simulink model "FMS"  (R2018b)
settings: configuration reference "fms_config" (kept outside this file)
values from neighbouring files (symbols this model uses):
  FMS_EXPORT = Simulink.Parameter(FMS_EXPORT_VALUE)    [fms_model_init.m]
  FMS_PARAM = Simulink.Parameter(FMS_PARAM_VALUE)    [fms_model_init.m]
undefined symbols (not defined in the file or in its folder): actuator_cmd, ay_cmd, cmd_mask, ControlMode, ctrl_mode, DiscIntNeverNeededParam, FMS_Cmd, mode, PilotMode, r_cmd, reset, state, status, theta_cmd, timestamp, u_cmd, VehicleState, VehicleStatus, w_cmd, wp_consume, wp_current
libraries: simulink x27, FMT_Model_Lib x21, hdlsllib x4
(part 1 of 3)
settings Model: Creator=jc  LastModifiedBy=zouji
settings ConfigSetRef: SourceLocation=Base Workspace

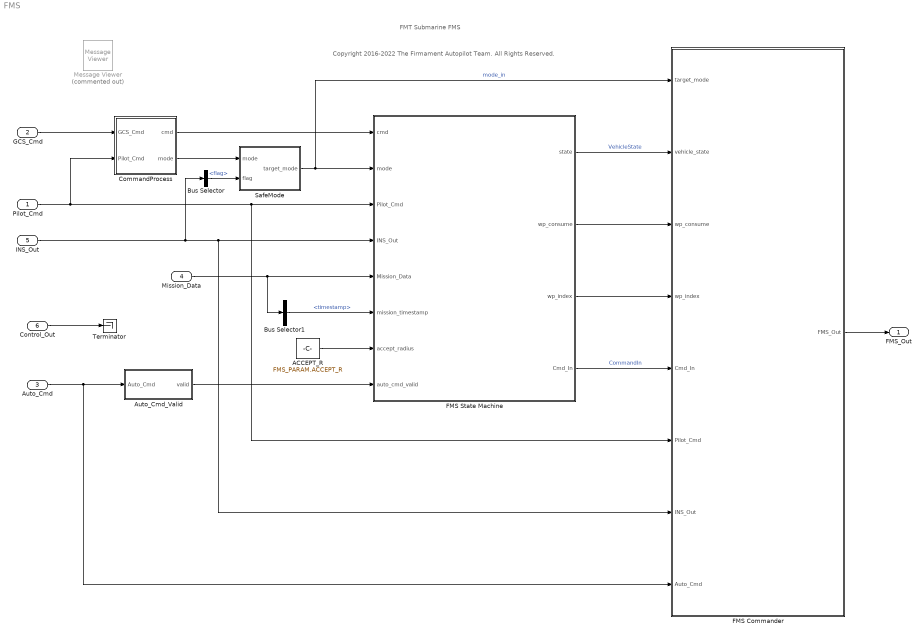
== system FMS ==
  note: Copyright 2016-2022 The Firmament Autopilot Team. All Rights Reserved.
  note: FMT Submarine FMS
  Pilot_Cmd : Inport  OutDataTypeStr=Bus: Pilot_Cmd_Bus
  GCS_Cmd : Inport  Port=2  OutDataTypeStr=Bus: GCS_Cmd_Bus
  Auto_Cmd : Inport  Port=3  OutDataTypeStr=Bus: Auto_Cmd_Bus
  Mission_Data : Inport  Port=4  OutDataTypeStr=Bus: Mission_Data_Bus  BusOutputAsStruct=on
  INS_Out : Inport  Port=5  OutDataTypeStr=Bus: INS_Out_Bus
  Control_Out : Inport  Port=6  OutDataTypeStr=Bus: Control_Out_Bus
  ACCEPT_R : Constant  Value=FMS_PARAM.ACCEPT_R
  Auto_Cmd_Valid : Subsystem
  Bus Selector : BusSelector  OutputSignals=flag
  Bus Selector1 : BusSelector  OutputSignals=timestamp
  CommandProcess : Subsystem  TreatAsAtomicUnit=on
  FMS Commander : Subsystem  TreatAsAtomicUnit=on
  FMS State Machine : Stateflow chart  TreatAsAtomicUnit=on
  Message Viewer : MessageViewer  Commented=on  SavedRootId=#
  SafeMode : Stateflow chart  TreatAsAtomicUnit=on
  Terminator : Terminator
  FMS_Out : Outport  OutDataTypeStr=Bus: FMS_Out_Bus
  wires:
  Control_Out/1 -> Terminator/1
  CommandProcess/1(cmd) -> FMS State Machine/1(cmd)
  FMS State Machine/4(Cmd_In) -> FMS Commander/5(Cmd_In)  "CommandIn"
  Auto_Cmd/1 -> Auto_Cmd_Valid/1(Auto_Cmd), FMS Commander/8(Auto_Cmd)
  Pilot_Cmd/1 -> FMS Commander/6(Pilot_Cmd), FMS State Machine/3(Pilot_Cmd), CommandProcess/2(Pilot_Cmd)
  INS_Out/1 -> Bus Selector/1, FMS Commander/7(INS_Out), FMS State Machine/4(INS_Out)
  CommandProcess/2(mode) -> SafeMode/1(mode)
  FMS Commander/1(FMS_Out) -> FMS_Out/1
  Bus Selector/1 -> SafeMode/2(flag)  "<flag>"
  GCS_Cmd/1 -> CommandProcess/1(GCS_Cmd)
  SafeMode/1(target_mode) -> FMS Commander/1(target_mode), FMS State Machine/2(mode)  "mode_in"
  FMS State Machine/1(state) -> FMS Commander/2(vehicle_state)  "VehicleState"
  Mission_Data/1 -> Bus Selector1/1, FMS State Machine/5(Mission_Data)
  FMS State Machine/2(wp_consume) -> FMS Commander/3(wp_consume)
  Bus Selector1/1 -> FMS State Machine/6(mission_timestamp)  "<timestamp>"
  FMS State Machine/3(wp_index) -> FMS Commander/4(wp_index)
  ACCEPT_R/1 -> FMS State Machine/7(accept_radius)
  Auto_Cmd_Valid/1(valid) -> FMS State Machine/8(auto_cmd_valid)

== system FMS/Auto_Cmd_Valid ==
  Auto_Cmd : Inport
  Bus Selector1 : BusSelector  OutputSignals=frame
  Bus Selector2 : BusSelector  OutputSignals=timestamp
  Compare To Constant4 : simulink/Logic and Bit Operations/Compare To Constant  relop=<  const=1000  OutDataTypeStr=boolean
  Constant : Constant  Value=FMS_EXPORT.period  OutDataTypeStr=single
  Detect Change : simulink/Logic and Bit Operations/Detect Change  vinit=0  OutDataTypeStr=boolean
  Discrete-Time Integrator : DiscreteIntegrator  IntegratorMethod=Accumulation: Forward Euler  ExternalReset=sampled level  SampleTime=-1  OutDataTypeStr=uint32  SaturateOnIntegerOverflow=on  ICPrevOutput=DiscIntNeverNeededParam  ICPrevScaledInput=DiscIntNeverNeededParam
  Ever_Valid : Subsystem
  Interval Test : simulink/Logic and Bit Operations/Interval Test  IntervalClosedRight=on  uplimit=2  IntervalClosedLeft=on  lowlimit=0  OutDataTypeStr=boolean
  Logical Operator : Logic  Inputs=3  AllPortsSameDT=off  OutDataTypeStr=boolean
  valid : Outport
  wires:
  Constant/1 -> Discrete-Time Integrator/1
  Detect Change/1 -> Ever_Valid/1(in), Discrete-Time Integrator/2
  Discrete-Time Integrator/1 -> Compare To Constant4/1
  Auto_Cmd/1 -> Bus Selector1/1, Bus Selector2/1
  Compare To Constant4/1 -> Logical Operator/1
  Ever_Valid/1(out) -> Logical Operator/2
  Logical Operator/1 -> valid/1
  Bus Selector2/1 -> Detect Change/1  "<timestamp>"
  Bus Selector1/1 -> Interval Test/1  "<frame>"
  Interval Test/1 -> Logical Operator/3

== system FMS/CommandProcess ==
  GCS_Cmd : Inport
  Pilot_Cmd : Inport  Port=2
  Check Valid : Subsystem
  Command Routing : Subsystem
  Mode Routing : Subsystem
  cmd : Outport
  mode : Outport  Port=2
  wires:
  GCS_Cmd/1 -> Mode Routing/2(GCS_Cmd), Command Routing/1(gcs_cmd)
  Pilot_Cmd/1 -> Command Routing/2(pilot_cmd), Check Valid/1(Pilot_Cmd), Mode Routing/3(Pilot_Cmd)
  Command Routing/1(cmd) -> cmd/1
  Check Valid/1(pilot_cmd_valid) -> Mode Routing/1(pilot_cmd_valid)
  Mode Routing/1(mode) -> mode/1  "fms_mode"

== system FMS/FMS Commander ==
  target_mode : Inport
  vehicle_state : Inport  Port=2
  wp_consume : Inport  Port=3
  wp_index : Inport  Port=4
  Cmd_In : Inport  Port=5
  Pilot_Cmd : Inport  Port=6
  INS_Out : Inport  Port=7
  Auto_Cmd : Inport  Port=8
  Commander : Subsystem
  FMS_Input : Subsystem  TreatAsAtomicUnit=on
  FMS_Out : Outport
  wires:
  target_mode/1 -> Commander/1(target_mode)
  FMS_Input/1(FMS_In) -> Commander/2(FMS_In)  "FMS_In"
  Commander/1(FMS_Out) -> FMS_Out/1
  vehicle_state/1 -> FMS_Input/1(state)
  wp_consume/1 -> FMS_Input/2(wp_consume)
  wp_index/1 -> FMS_Input/3(wp_index)
  Cmd_In/1 -> FMS_Input/4(Cmd_In)
  Pilot_Cmd/1 -> FMS_Input/5(Pilot_Cmd)
  INS_Out/1 -> FMS_Input/6(INS_Out)
  Auto_Cmd/1 -> FMS_Input/7(Auto_Cmd)

== system FMS/FMS State Machine/Vehicle.Arm.Auto.Mission.LLA2FLAT ==
  lla : Inport  OutDataTypeStr=double  PortDimensions=[1 3]
  llo : Inport  Port=2  OutDataTypeStr=double  Unit=deg  PortDimensions=[1 2]
  href : Inport  Port=3  OutDataTypeStr=double  Unit=m  PortDimensions=1
  psio : Inport  Port=4  OutDataTypeStr=double  Unit=deg  PortDimensions=1
  f : TriggerPort  TriggerType=function-call  VariantControl=(inherit)
      settings: CopyFcn=Stateflow.SLINSF.SimulinkMan.removeBlockPreDeleteFcn  PreDeleteFcn=Stateflow.SLINSF.SimulinkMan.unsafePredeleteFcn
  Data Type Conversion : DataTypeConversion  OutDataTypeStr=single
  LLA2FLAT : FMT_Model_Lib/Transformation/LLA2FLAT
      settings: SourceProductName=FMT Toolbox
  Signal Conversion : SignalConversion  OverrideOpt=off
  pos : Outport
  wires:
  LLA2FLAT/1 -> Signal Conversion/1
  lla/1 -> LLA2FLAT/1
  llo/1 -> LLA2FLAT/2
  href/1 -> LLA2FLAT/3
  psio/1 -> LLA2FLAT/4
  Signal Conversion/1 -> Data Type Conversion/1
  Data Type Conversion/1 -> pos/1

== system FMS/FMS State Machine/Vehicle.StickMoved ==
  stick_val : Inport  OutDataTypeStr=double  PortDimensions=4
  pilot_cmd : Inport  Port=2  OutDataTypeStr=Bus: Pilot_Cmd_Bus  PortDimensions=1
  f : TriggerPort  TriggerType=function-call  VariantControl=(inherit)
      settings: CopyFcn=Stateflow.SLINSF.SimulinkMan.removeBlockPreDeleteFcn  PreDeleteFcn=Stateflow.SLINSF.SimulinkMan.unsafePredeleteFcn
  Abs : Abs
  Bus Selector : BusSelector  OutputSignals=stick_yaw,stick_throttle,stick_roll,stick_pitch
  Compare To Constant : simulink/Logic and Bit Operations/Compare To Constant  relop=>=  const=0.1  OutDataTypeStr=boolean
  Max : MinMax  Function=max
  Mux : Mux
  Sum : Sum  Inputs=|+-
  moved : Outport
  wires:
  pilot_cmd/1 -> Bus Selector/1
  Bus Selector/1 -> Mux/1  "<stick_yaw>"
  Bus Selector/2 -> Mux/2  "<stick_throttle>"
  Bus Selector/3 -> Mux/3  "<stick_roll>"
  Bus Selector/4 -> Mux/4  "<stick_pitch>"
  stick_val/1 -> Sum/1
  Mux/1 -> Sum/2
  Sum/1 -> Abs/1
  Abs/1 -> Max/1
  Max/1 -> Compare To Constant/1
  Compare To Constant/1 -> moved/1

== system FMS/Auto_Cmd_Valid/Ever_Valid ==
  in : Inport
  Constant1 : Constant  OutDataTypeStr=uint8
  Delay : Delay  DelayLength=1
  Switch : Switch  Criteria=u2 > Threshold
  out : Outport
  wires:
  Constant1/1 -> Switch/1
  Delay/1 -> Switch/3
  in/1 -> Switch/2
  Switch/1 -> out/1, Delay/1

== system FMS/CommandProcess/Check Valid ==
  Pilot_Cmd : Inport
  Bus Selector1 : BusSelector  OutputSignals=timestamp
  Compare To Constant1 : simulink/Logic and Bit Operations/Compare To Constant  relop=<  const=500  OutDataTypeStr=boolean
  Constant1 : Constant  Value=FMS_EXPORT.period  OutDataTypeStr=single
  Detect Change1 : simulink/Logic and Bit Operations/Detect Change  vinit=0  OutDataTypeStr=boolean
  Discrete-Time Integrator1 : DiscreteIntegrator  IntegratorMethod=Accumulation: Forward Euler  ExternalReset=sampled level  SampleTime=-1  OutDataTypeStr=uint32  SaturateOnIntegerOverflow=on  ICPrevOutput=DiscIntNeverNeededParam  ICPrevScaledInput=DiscIntNeverNeededParam
  pilot_cmd_valid : Outport
  wires:
  Pilot_Cmd/1 -> Bus Selector1/1
  Compare To Constant1/1 -> pilot_cmd_valid/1
  Bus Selector1/1 -> Detect Change1/1  "<timestamp>"
  Constant1/1 -> Discrete-Time Integrator1/1
  Detect Change1/1 -> Discrete-Time Integrator1/2
  Discrete-Time Integrator1/1 -> Compare To Constant1/1

== system FMS/CommandProcess/Command Routing ==
  gcs_cmd : Inport
  pilot_cmd : Inport  Port=2
  Bus Selector : BusSelector  OutputSignals=cmd_1
  Bus Selector1 : BusSelector  OutputSignals=cmd_1
  Constant1 : Constant  Value=FMS_Cmd.None
  Data Type Conversion1 : DataTypeConversion  OutDataTypeStr=Enum: FMS_Cmd
  Data Type Conversion2 : DataTypeConversion  OutDataTypeStr=Enum: FMS_Cmd
  Detect Change3 : simulink/Logic and Bit Operations/Detect Change  vinit=0  OutDataTypeStr=boolean
  Detect Change4 : simulink/Logic and Bit Operations/Detect Change  vinit=0  OutDataTypeStr=boolean
  Switch1 : Switch  Criteria=u2 > Threshold
  Switch2 : Switch  Criteria=u2 > Threshold
  cmd : Outport
  wires:
  Bus Selector/1 -> Data Type Conversion1/1, Detect Change4/1  "<cmd_1>"
  pilot_cmd/1 -> Bus Selector1/1
  Switch1/1 -> cmd/1
  gcs_cmd/1 -> Bus Selector/1
  Bus Selector1/1 -> Data Type Conversion2/1, Detect Change3/1  "<cmd_1>"
  Detect Change3/1 -> Switch1/2
  Switch2/1 -> Switch1/3
  Detect Change4/1 -> Switch2/2
  Data Type Conversion2/1 -> Switch1/1
  Data Type Conversion1/1 -> Switch2/1
  Constant1/1 -> Switch2/3

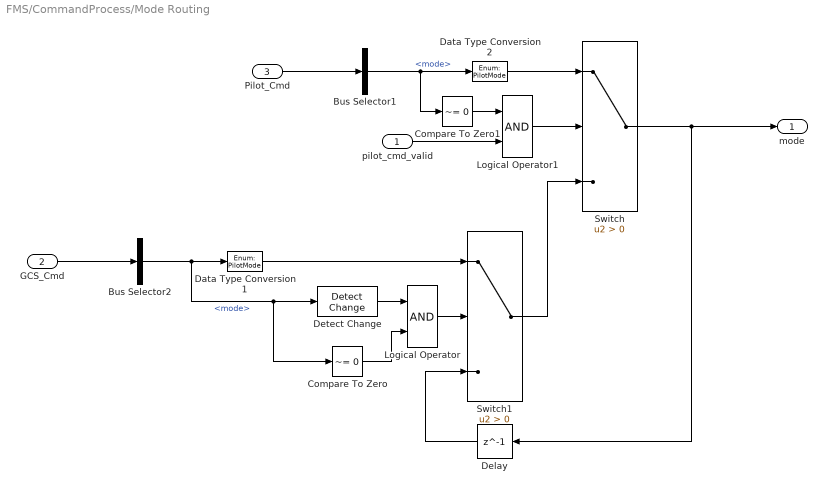
== system FMS/CommandProcess/Mode Routing ==
  pilot_cmd_valid : Inport
  GCS_Cmd : Inport  Port=2
  Pilot_Cmd : Inport  Port=3
  Bus Selector1 : BusSelector  OutputSignals=mode
  Bus Selector2 : BusSelector  OutputSignals=mode
  Compare To Zero : simulink/Logic and Bit Operations/Compare To Zero  relop=~=  OutDataTypeStr=boolean
  Compare To Zero1 : simulink/Logic and Bit Operations/Compare To Zero  relop=~=  OutDataTypeStr=boolean
  Data Type Conversion1 : DataTypeConversion  OutDataTypeStr=Enum: PilotMode
  Data Type Conversion2 : DataTypeConversion  OutDataTypeStr=Enum: PilotMode
  Delay : Delay  DelayLength=1  InitialCondition=PilotMode.None
  Detect Change : simulink/Logic and Bit Operations/Detect Change  vinit=0  OutDataTypeStr=boolean
  Logical Operator : Logic  AllPortsSameDT=off  OutDataTypeStr=boolean
  Logical Operator1 : Logic  AllPortsSameDT=off  OutDataTypeStr=boolean
  Switch : Switch  Criteria=u2 > Threshold
  Switch1 : Switch  Criteria=u2 > Threshold
  mode : Outport
  wires:
  Bus Selector2/1 -> Compare To Zero/1, Detect Change/1, Data Type Conversion1/1  "<mode>"
  GCS_Cmd/1 -> Bus Selector2/1
  Pilot_Cmd/1 -> Bus Selector1/1
  Bus Selector1/1 -> Compare To Zero1/1, Data Type Conversion2/1  "<mode>"
  Logical Operator1/1 -> Switch/2
  Data Type Conversion2/1 -> Switch/1
  Switch/1 -> mode/1, Delay/1
  Delay/1 -> Switch1/3
  Compare To Zero/1 -> Logical Operator/2
  Data Type Conversion1/1 -> Switch1/1
  Switch1/1 -> Switch/3
  Detect Change/1 -> Logical Operator/1
  Logical Operator/1 -> Switch1/2
  pilot_cmd_valid/1 -> Logical Operator1/2
  Compare To Zero1/1 -> Logical Operator1/1

== system FMS/FMS Commander/Commander ==
  target_mode : Inport
  FMS_In : Inport  Port=2
  Arm : Subsystem  TreatAsAtomicUnit=on
  Bus Selector1 : BusSelector  OutputSignals=vehicle_state
  Bus_Constructor : Subsystem
  Disarm : Subsystem  TreatAsAtomicUnit=on
  FMS_In1 : InportShadow  Port=2
  FMS_In2 : InportShadow  Port=2
  Merge : Merge  Inputs=3
  Standby : Subsystem  TreatAsAtomicUnit=on
  Switch Case : SwitchCase  CaseConditions={[VehicleState.Disarm,VehicleState.None], VehicleState.Standby}
  FMS_Out : Outport
  wires:
  Switch Case/3 -> Arm/Action
  Bus Selector1/1 -> Switch Case/1  "<vehicle_state>"
  FMS_In/1 -> Bus Selector1/1
  Standby/1(FMS_Out) -> Merge/2
  Arm/1(FMS_Out) -> Merge/3
  Switch Case/2 -> Standby/Action
  Switch Case/1 -> Disarm/Action
  Disarm/1(FMS_Out) -> Merge/1
  FMS_In1/1 -> Arm/1(FMS_In)
  Merge/1 -> Bus_Constructor/1(Bus_In)
  target_mode/1 -> Bus_Constructor/2(target_mode)
  FMS_In2/1 -> Bus_Constructor/3(FMS_In)
  Bus_Constructor/1(FMS_Out) -> FMS_Out/1

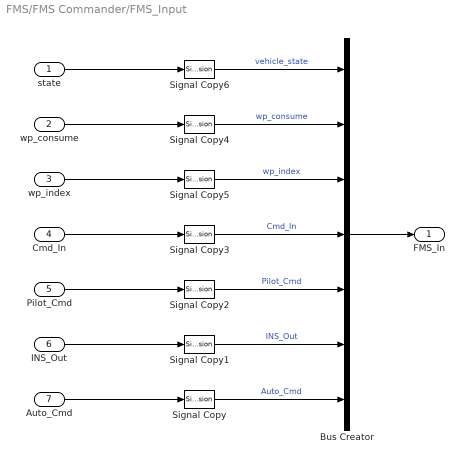
== system FMS/FMS Commander/FMS_Input ==
  state : Inport
  wp_consume : Inport  Port=2
  wp_index : Inport  Port=3
  Cmd_In : Inport  Port=4
  Pilot_Cmd : Inport  Port=5
  INS_Out : Inport  Port=6
  Auto_Cmd : Inport  Port=7
  Bus Creator : BusCreator  Inputs=7
  Signal Copy{,1..6} (7 alike) : SignalConversion  OverrideOpt=off
  FMS_In : Outport
  wires:
  Bus Creator/1 -> FMS_In/1
  Pilot_Cmd/1 -> Signal Copy2/1
  Auto_Cmd/1 -> Signal Copy/1
  INS_Out/1 -> Signal Copy1/1
  Signal Copy2/1 -> Bus Creator/5  "Pilot_Cmd"
  Signal Copy/1 -> Bus Creator/7  "Auto_Cmd"
  Signal Copy1/1 -> Bus Creator/6  "INS_Out"
  Cmd_In/1 -> Signal Copy3/1
  Signal Copy3/1 -> Bus Creator/4  "Cmd_In"
  wp_index/1 -> Signal Copy5/1
  Signal Copy5/1 -> Bus Creator/3  "wp_index"
  wp_consume/1 -> Signal Copy4/1
  Signal Copy4/1 -> Bus Creator/2  "wp_consume"
  state/1 -> Signal Copy6/1
  Signal Copy6/1 -> Bus Creator/1  "vehicle_state"

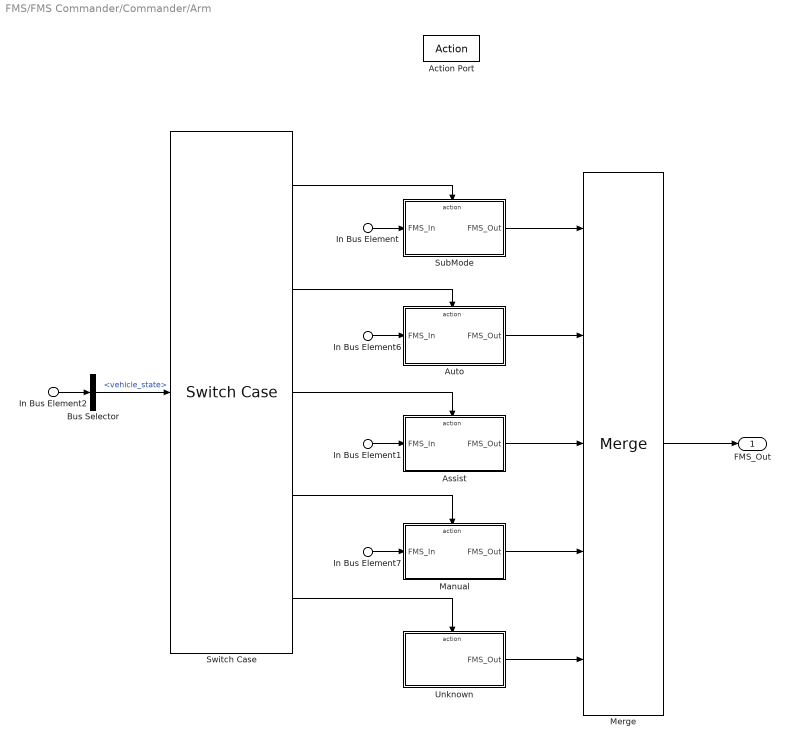
== system FMS/FMS Commander/Commander/Arm ==
  In Bus Element{,1..2,6..7} (5 alike) : Inport  PortName=FMS_In
  Action Port : ActionPort  InitializeStates=reset  ActionType=default
  Assist : Subsystem  TreatAsAtomicUnit=on
  Auto : Subsystem  TreatAsAtomicUnit=on
  Bus Selector : BusSelector  OutputSignals=vehicle_state
  Manual : Subsystem  TreatAsAtomicUnit=on
  Merge : Merge  Inputs=5
  SubMode : Subsystem  TreatAsAtomicUnit=on
  Switch Case : SwitchCase  CaseConditions={[VehicleState.Land,VehicleState.Return,VehicleState.Takeoff,VehicleState.Hold], [VehicleState.Offboard,VehicleState.Mission],[VehicleState.Acro,VehicleState.Stabilize,VehicleState.Altitude,VehicleState.Position],VehicleState.Manual}
  Unknown : Subsystem  TreatAsAtomicUnit=on
  FMS_Out : Outport
  wires:
  Merge/1 -> FMS_Out/1
  Switch Case/1 -> SubMode/Action
  Switch Case/2 -> Auto/Action
  Switch Case/3 -> Assist/Action
  Switch Case/4 -> Manual/Action
  SubMode/1(FMS_Out) -> Merge/1
  Auto/1(FMS_Out) -> Merge/2
  Assist/1(FMS_Out) -> Merge/3
  Manual/1(FMS_Out) -> Merge/4
  In Bus Element/1 -> SubMode/1(FMS_In)
  In Bus Element1/1 -> Assist/1(FMS_In)
  In Bus Element6/1 -> Auto/1(FMS_In)
  In Bus Element7/1 -> Manual/1(FMS_In)
  Switch Case/5 -> Unknown/Action
  Unknown/1(FMS_Out) -> Merge/5
  In Bus Element2/1 -> Bus Selector/1
  Bus Selector/1 -> Switch Case/1  "<vehicle_state>"

== system FMS/FMS Commander/Commander/Bus_Constructor ==
  Bus_In : Inport
  target_mode : Inport  Port=2
  FMS_In : Inport  Port=3
  Bus Assignment : BusAssignment  AssignedSignals=timestamp,mode,wp_consume,wp_current
  Bus Selector : BusSelector  OutputSignals=wp_consume,wp_index
  Constant : Constant  OutDataTypeStr=uint8
  Data Type Conversion : DataTypeConversion
  Sum : Sum  Inputs=|+-
  timestamp : Subsystem  mask{sample_time=FMS_EXPORT.period}
      mask prompts: sample_time "sample time (ms)"
  FMS_Out : Outport
  wires:
  Sum/1 -> Bus Assignment/5
  Bus Selector/1 -> Bus Assignment/4  "<wp_consume>"
  Bus Selector/2 -> Sum/1  "<wp_index>"
  Constant/1 -> Sum/2
  target_mode/1 -> Data Type Conversion/1
  Bus_In/1 -> Bus Assignment/1
  Bus Assignment/1 -> FMS_Out/1
  Data Type Conversion/1 -> Bus Assignment/3
  FMS_In/1 -> Bus Selector/1
  timestamp/1(timestamp_ms) -> Bus Assignment/2

== system FMS/FMS Commander/Commander/Disarm ==
  Action Port : ActionPort  InitializeStates=reset  ActionType=case
  Bus Assignment : BusAssignment  AssignedSignals=reset,status,state
  Constant : Constant  Value=0  OutDataTypeStr=Bus: FMS_Out_Bus
  Constant1 : Constant  Value=VehicleStatus.Disarm
  Constant2 : Constant  OutDataTypeStr=Inherit: Inherit via back propagation
  Constant5 : Constant  Value=VehicleState.Disarm
  Data Type Conversion : DataTypeConversion
  Data Type Conversion1 : DataTypeConversion
  FMS_Out : Outport
  wires:
  Constant1/1 -> Data Type Conversion/1
  Constant2/1 -> Bus Assignment/2
  Bus Assignment/1 -> FMS_Out/1
  Constant/1 -> Bus Assignment/1
  Constant5/1 -> Data Type Conversion1/1
  Data Type Conversion/1 -> Bus Assignment/3
  Data Type Conversion1/1 -> Bus Assignment/4

== system FMS/FMS Commander/Commander/Standby ==
  Action Port : ActionPort  InitializeStates=reset  ActionType=case
  Bus Assignment : BusAssignment  AssignedSignals=reset,status,state
  Constant : Constant  Value=0  OutDataTypeStr=Bus: FMS_Out_Bus
  Constant1 : Constant  Value=VehicleStatus.Standby
  Constant2 : Constant  OutDataTypeStr=Inherit: Inherit via back propagation
  Constant5 : Constant  Value=VehicleState.Standby
  Data Type Conversion1 : DataTypeConversion
  Data Type Conversion2 : DataTypeConversion
  FMS_Out : Outport
  wires:
  Constant/1 -> Bus Assignment/1
  Bus Assignment/1 -> FMS_Out/1
  Constant2/1 -> Bus Assignment/2
  Constant1/1 -> Data Type Conversion2/1
  Constant5/1 -> Data Type Conversion1/1
  Data Type Conversion2/1 -> Bus Assignment/3
  Data Type Conversion1/1 -> Bus Assignment/4

== system FMS/FMS Commander/Commander/Arm/Assist ==
  In Bus Element{1..3,5} (4 alike) : Inport  PortName=FMS_In
  Action Port : ActionPort  InitializeStates=reset  ActionType=case
  Altitude : Subsystem
      settings: UndoDeleteFcn=Stateflow.SLINSF.SimulinkMan.restorePreDeleteFcn  PreDeleteFcn=Stateflow.SLINSF.SimulinkMan.removePreDeleteFcn
  Bus Selector : BusSelector  OutputSignals=vehicle_state
  Merge : Merge  Inputs=4
  Position : Subsystem
      settings: UndoDeleteFcn=Stateflow.SLINSF.SimulinkMan.restorePreDeleteFcn  PreDeleteFcn=Stateflow.SLINSF.SimulinkMan.removePreDeleteFcn
  Stabilize : Subsystem
      settings: UndoDeleteFcn=Stateflow.SLINSF.SimulinkMan.restorePreDeleteFcn  PreDeleteFcn=Stateflow.SLINSF.SimulinkMan.removePreDeleteFcn
  Switch Case : SwitchCase  CaseConditions={VehicleState.Stabilize,VehicleState.Altitude,VehicleState.Position}
  Unknown : Subsystem  TreatAsAtomicUnit=on
  FMS_Out : Outport
  wires:
  In Bus Element3/1 -> Position/1(FMS_In)
  In Bus Element2/1 -> Altitude/1(FMS_In)
  In Bus Element1/1 -> Stabilize/1(FMS_In)
  Merge/1 -> FMS_Out/1
  In Bus Element5/1 -> Bus Selector/1
  Bus Selector/1 -> Switch Case/1  "<vehicle_state>"
  Stabilize/1(FMS_Out) -> Merge/1
  Altitude/1(FMS_Out) -> Merge/2
  Position/1(FMS_Out) -> Merge/3
  Unknown/1(FMS_Out) -> Merge/4
  Switch Case/1 -> Stabilize/Action
  Switch Case/2 -> Altitude/Action
  Switch Case/3 -> Position/Action
  Switch Case/4 -> Unknown/Action

== system FMS/FMS Commander/Commander/Arm/Auto ==
  In Bus Element6 : Inport  PortName=FMS_In
  In Bus Element1 : Inport  PortName=FMS_In
  In Bus Element2 : Inport  PortName=FMS_In
  Action Port : ActionPort  InitializeStates=reset  ActionType=case
  Bus Selector : BusSelector  OutputSignals=vehicle_state
  Merge : Merge  Inputs=3
  Mission : Subsystem
      settings: UndoDeleteFcn=Stateflow.SLINSF.SimulinkMan.restorePreDeleteFcn  PreDeleteFcn=Stateflow.SLINSF.SimulinkMan.removePreDeleteFcn
  Offboard : Subsystem
      settings: UndoDeleteFcn=Stateflow.SLINSF.SimulinkMan.restorePreDeleteFcn  PreDeleteFcn=Stateflow.SLINSF.SimulinkMan.removePreDeleteFcn
  Switch Case : SwitchCase  CaseConditions={VehicleState.Offboard,VehicleState.Mission}
  Unknown : Subsystem  TreatAsAtomicUnit=on
  FMS_Out : Outport
  wires:
  Merge/1 -> FMS_Out/1
  In Bus Element6/1 -> Offboard/1(FMS_In)
  Switch Case/1 -> Offboard/Action
  In Bus Element1/1 -> Mission/1(FMS_In)
  Switch Case/2 -> Mission/Action
  Offboard/1(FMS_Out) -> Merge/1
  Mission/1(FMS_Out) -> Merge/2
  Unknown/1(FMS_Out) -> Merge/3
  Switch Case/3 -> Unknown/Action
  In Bus Element2/1 -> Bus Selector/1
  Bus Selector/1 -> Switch Case/1  "<vehicle_state>"

== system FMS/FMS Commander/Commander/Arm/Manual ==
  In Bus Element7 : Inport  PortName=FMS_In
  Action Port : ActionPort  InitializeStates=reset  ActionType=case
  Bus Assignment : BusAssignment  AssignedSignals=reset,status,state
  Constant : Constant  Value=0  OutDataTypeStr=Bus: FMS_Out_Bus
  Constant1 : Constant  Value=VehicleStatus.Disarm
  Constant2 : Constant  OutDataTypeStr=Inherit: Inherit via back propagation
  Constant5 : Constant  Value=VehicleState.Manual
  Data Type Conversion : DataTypeConversion
  Data Type Conversion1 : DataTypeConversion
  Terminator : Terminator
  FMS_Out : Outport
  wires:
  Data Type Conversion1/1 -> Bus Assignment/4
  Data Type Conversion/1 -> Bus Assignment/3
  Constant5/1 -> Data Type Conversion1/1
  Constant/1 -> Bus Assignment/1
  Bus Assignment/1 -> FMS_Out/1
  Constant2/1 -> Bus Assignment/2
  Constant1/1 -> Data Type Conversion/1
  In Bus Element7/1 -> Terminator/1

== system FMS/FMS Commander/Commander/Arm/SubMode ==
  In Bus Element5 : Inport  PortName=FMS_In
  In Bus Element1 : Inport  PortName=FMS_In
  In Bus Element2 : Inport  PortName=FMS_In
  Action Port : ActionPort  InitializeStates=reset  ActionType=case
  Bus Selector : BusSelector  OutputSignals=vehicle_state
  Hold : Subsystem
      settings: UndoDeleteFcn=Stateflow.SLINSF.SimulinkMan.restorePreDeleteFcn  PreDeleteFcn=Stateflow.SLINSF.SimulinkMan.removePreDeleteFcn
  Merge : Merge  Inputs=3
  Return : Subsystem
      settings: UndoDeleteFcn=Stateflow.SLINSF.SimulinkMan.restorePreDeleteFcn  PreDeleteFcn=Stateflow.SLINSF.SimulinkMan.removePreDeleteFcn
  Switch Case : SwitchCase  CaseConditions={VehicleState.Return, VehicleState.Hold}
  Unknown : Subsystem  TreatAsAtomicUnit=on
  FMS_Out : Outport
  wires:
  Merge/1 -> FMS_Out/1
  In Bus Element1/1 -> Return/1(FMS_In)
  Return/1(FMS_Out) -> Merge/1
  Unknown/1(FMS_Out) -> Merge/3
  In Bus Element5/1 -> Bus Selector/1
  Bus Selector/1 -> Switch Case/1  "<vehicle_state>"
  In Bus Element2/1 -> Hold/1(FMS_In)
  Hold/1(FMS_Out) -> Merge/2
  Switch Case/1 -> Return/Action
  Switch Case/2 -> Hold/Action
  Switch Case/3 -> Unknown/Action

== system FMS/FMS Commander/Commander/Arm/Unknown ==
  Action Port : ActionPort  InitializeStates=reset  ActionType=default
  Bus Assignment : BusAssignment  AssignedSignals=reset,status,state,actuator_cmd
  Constant : Constant  Value=0  OutDataTypeStr=Bus: FMS_Out_Bus
  Constant1 : Constant  Value=VehicleStatus.Disarm
  Constant2 : Constant  OutDataTypeStr=Inherit: Inherit via back propagation
  Constant3 : Constant  Value=[1000;1000;1000;1000]  VectorParams1D=off  OutDataTypeStr=Inherit: Inherit via back propagation
  Constant4 : Constant  Value=zeros(12,1)  OutDataTypeStr=Inherit: Inherit via back propagation
  Constant5 : Constant  Value=VehicleState.Disarm
  Data Type Conversion : DataTypeConversion
  Data Type Conversion1 : DataTypeConversion
  Mux : Mux  Inputs=2
  FMS_Out : Outport
  wires:
  Mux/1 -> Bus Assignment/5
  Constant4/1 -> Mux/2
  Constant3/1 -> Mux/1
  Constant1/1 -> Data Type Conversion/1
  Constant2/1 -> Bus Assignment/2
  Bus Assignment/1 -> FMS_Out/1
  Constant/1 -> Bus Assignment/1
  Constant5/1 -> Data Type Conversion1/1
  Data Type Conversion/1 -> Bus Assignment/3
  Data Type Conversion1/1 -> Bus Assignment/4

== system FMS/FMS Commander/Commander/Bus_Constructor/timestamp ==
  Constant : Constant  Value=sample_time
  Data Type Conversion : DataTypeConversion  OutDataTypeStr=uint32
  Discrete-Time Integrator : DiscreteIntegrator  IntegratorMethod=Accumulation: Forward Euler  SampleTime=-1  ICPrevOutput=DiscIntNeverNeededParam  ICPrevScaledInput=DiscIntNeverNeededParam
  timestamp_ms : Outport
  wires:
  Discrete-Time Integrator/1 -> Data Type Conversion/1
  Constant/1 -> Discrete-Time Integrator/1
  Data Type Conversion/1 -> timestamp_ms/1

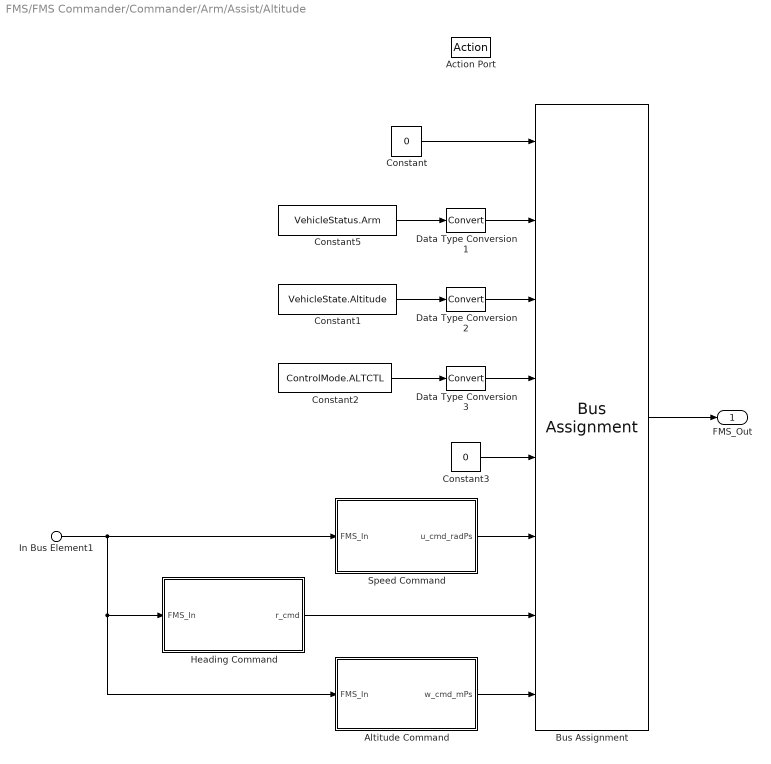
== system FMS/FMS Commander/Commander/Arm/Assist/Altitude ==
  In Bus Element1 : Inport  PortName=FMS_In
  Action Port : ActionPort  InitializeStates=reset  ActionType=case
      settings: CopyFcn=Stateflow.SLINSF.SimulinkMan.removeBlockPreDeleteFcn
  Altitude Command : Subsystem
  Bus Assignment : BusAssignment  AssignedSignals=status,state,ctrl_mode,theta_cmd,u_cmd,r_cmd,w_cmd
  Constant : Constant  Value=0  OutDataTypeStr=Bus: FMS_Out_Bus
  Constant1 : Constant  Value=VehicleState.Altitude
  Constant2 : Constant  Value=ControlMode.ALTCTL
  Constant3 : Constant  Value=0  OutDataTypeStr=single
  Constant5 : Constant  Value=VehicleStatus.Arm
  Data Type Conversion1 : DataTypeConversion
  Data Type Conversion2 : DataTypeConversion
  Data Type Conversion3 : DataTypeConversion
  Heading Command : Subsystem
  Speed Command : Subsystem
  FMS_Out : Outport
  wires:
  Constant5/1 -> Data Type Conversion1/1
  Constant/1 -> Bus Assignment/1
  Bus Assignment/1 -> FMS_Out/1
  Data Type Conversion1/1 -> Bus Assignment/2
  Constant1/1 -> Data Type Conversion2/1
  Data Type Conversion2/1 -> Bus Assignment/3
  Data Type Conversion3/1 -> Bus Assignment/4
  Constant2/1 -> Data Type Conversion3/1
  Speed Command/1(u_cmd_radPs) -> Bus Assignment/6
  In Bus Element1/1 -> Heading Command/1(FMS_In), Altitude Command/1(FMS_In), Speed Command/1(FMS_In)
  Altitude Command/1(w_cmd_mPs) -> Bus Assignment/8
  Heading Command/1(r_cmd) -> Bus Assignment/7
  Constant3/1 -> Bus Assignment/5

== system FMS/FMS Commander/Commander/Arm/Assist/Position ==
  FMS_In : Inport
  Action Port : ActionPort  InitializeStates=reset  ActionType=case
      settings: CopyFcn=Stateflow.SLINSF.SimulinkMan.removeBlockPreDeleteFcn
  Altitude Command : Subsystem
  Bus Assignment : BusAssignment  AssignedSignals=status,state,ctrl_mode,theta_cmd,u_cmd,r_cmd,w_cmd
  Constant : Constant  Value=0  OutDataTypeStr=Bus: FMS_Out_Bus
  Constant1 : Constant  Value=VehicleState.Position
  Constant2 : Constant  Value=ControlMode.POSCTL
  Constant3 : Constant  Value=0  OutDataTypeStr=single
  Constant5 : Constant  Value=VehicleStatus.Arm
  Data Type Conversion : DataTypeConversion
  Data Type Conversion1 : DataTypeConversion
  Data Type Conversion2 : DataTypeConversion
  Heading Command : Subsystem
  Speed Command : Subsystem
  FMS_Out : Outport
  wires:
  Bus Assignment/1 -> FMS_Out/1
  Constant/1 -> Bus Assignment/1
  Constant5/1 -> Data Type Conversion/1
  Data Type Conversion/1 -> Bus Assignment/2
  Constant1/1 -> Data Type Conversion1/1
  Data Type Conversion1/1 -> Bus Assignment/3
  Constant2/1 -> Data Type Conversion2/1
  Data Type Conversion2/1 -> Bus Assignment/4
  Heading Command/1(r_cmd) -> Bus Assignment/7
  FMS_In/1 -> Altitude Command/1(FMS_In), Heading Command/1(FMS_In), Speed Command/1(FMS_In)
  Constant3/1 -> Bus Assignment/5
  Speed Command/1(u_cmd_radPs) -> Bus Assignment/6
  Altitude Command/1(w_cmd_mPs) -> Bus Assignment/8

== system FMS/FMS Commander/Commander/Arm/Assist/Stabilize ==
  FMS_In : Inport
  Action Port : ActionPort  InitializeStates=reset  ActionType=case
      settings: CopyFcn=Stateflow.SLINSF.SimulinkMan.removeBlockPreDeleteFcn
  "Altitude Command " : Subsystem
  Bus Assignment : BusAssignment  AssignedSignals=status,state,ctrl_mode,theta_cmd,u_cmd,r_cmd,w_cmd
  Constant : Constant  Value=0  OutDataTypeStr=Bus: FMS_Out_Bus
  Constant1 : Constant  Value=VehicleState.Stabilize
  Constant2 : Constant  Value=ControlMode.Stabilize
  Constant3 : Constant  Value=0  OutDataTypeStr=single
  Constant5 : Constant  Value=VehicleStatus.Arm
  Data Type Conversion : DataTypeConversion
  Data Type Conversion1 : DataTypeConversion
  Data Type Conversion2 : DataTypeConversion
  Heading Command : Subsystem
  Speed Command : Subsystem
  FMS_Out : Outport
  wires:
  Constant5/1 -> Data Type Conversion/1
  Constant/1 -> Bus Assignment/1
  FMS_In/1 -> "Altitude Command "/1(FMS_In), Heading Command/1(FMS_In), Speed Command/1(FMS_In)
  Bus Assignment/1 -> FMS_Out/1
  Data Type Conversion/1 -> Bus Assignment/2
  Constant1/1 -> Data Type Conversion1/1
  Data Type Conversion1/1 -> Bus Assignment/3
  Constant2/1 -> Data Type Conversion2/1
  Data Type Conversion2/1 -> Bus Assignment/4
  Heading Command/1(r_cmd) -> Bus Assignment/7
  Constant3/1 -> Bus Assignment/5
  Speed Command/1(u_cmd_radPs) -> Bus Assignment/6
  "Altitude Command "/1(w_cmd_mPs) -> Bus Assignment/8

== system FMS/FMS Commander/Commander/Arm/Assist/Unknown ==
  Action Port : ActionPort  InitializeStates=reset  ActionType=default
  Bus Assignment : BusAssignment  AssignedSignals=reset,status,state,actuator_cmd
  Constant : Constant  Value=0  OutDataTypeStr=Bus: FMS_Out_Bus
  Constant1 : Constant  Value=VehicleStatus.Disarm
  Constant2 : Constant  OutDataTypeStr=Inherit: Inherit via back propagation
  Constant3 : Constant  Value=[1000;1000;1000;1000]  VectorParams1D=off  OutDataTypeStr=Inherit: Inherit via back propagation
  Constant4 : Constant  Value=zeros(12,1)  OutDataTypeStr=Inherit: Inherit via back propagation
  Constant5 : Constant  Value=VehicleState.Disarm
  Data Type Conversion : DataTypeConversion
  Data Type Conversion1 : DataTypeConversion
  Mux : Mux  Inputs=2
  FMS_Out : Outport
  wires:
  Mux/1 -> Bus Assignment/5
  Constant4/1 -> Mux/2
  Constant3/1 -> Mux/1
  Constant1/1 -> Data Type Conversion/1
  Constant2/1 -> Bus Assignment/2
  Bus Assignment/1 -> FMS_Out/1
  Constant/1 -> Bus Assignment/1
  Constant5/1 -> Data Type Conversion1/1
  Data Type Conversion/1 -> Bus Assignment/3
  Data Type Conversion1/1 -> Bus Assignment/4

== system FMS/FMS Commander/Commander/Arm/Auto/Mission ==
  FMS_In : Inport
  Action Port : ActionPort  InitializeStates=reset  ActionType=case
      settings: CopyFcn=Stateflow.SLINSF.SimulinkMan.removeBlockPreDeleteFcn
  Bus Selector : BusSelector  OutputSignals=wp_index
  Detect Change : simulink/Logic and Bit Operations/Detect Change  vinit=0  OutDataTypeStr=boolean
  Mission_SubSystem : Subsystem  TreatAsAtomicUnit=on
  FMS_Out : Outport
  wires:
  Mission_SubSystem/1(FMS_Out) -> FMS_Out/1
  FMS_In/1 -> Bus Selector/1, Mission_SubSystem/1(FMS_In)
  Bus Selector/1 -> Detect Change/1  "<wp_index>"
  Detect Change/1 -> Mission_SubSystem/Reset

== system FMS/FMS Commander/Commander/Arm/Auto/Offboard ==
  FMS_In : Inport
  Action Port : ActionPort  InitializeStates=reset  ActionType=case
      settings: CopyFcn=Stateflow.SLINSF.SimulinkMan.removeBlockPreDeleteFcn
  Bus Assignment : BusAssignment  AssignedSignals=status,state,ctrl_mode,r_cmd,theta_cmd,u_cmd,w_cmd,cmd_mask
  Bus Selector1 : BusSelector  OutputSignals=Auto_Cmd.psi_rate_cmd,Auto_Cmd.theta_cmd,Auto_Cmd.u_cmd,Auto_Cmd.w_cmd
  Command_Mask : Subsystem
  Constant : Constant  Value=0  OutDataTypeStr=Bus: FMS_Out_Bus
  Constant1 : Constant  Value=VehicleStatus.Arm
  Constant2 : Constant  Value=VehicleState.Offboard
  Constant3 : Constant  Value=ControlMode.Offboard
  Data Type Conversion : DataTypeConversion
  Data Type Conversion1 : DataTypeConversion
  Data Type Conversion2 : DataTypeConversion
  FMS_Out : Outport
  wires:
  Bus Assignment/1 -> FMS_Out/1
  Constant2/1 -> Data Type Conversion1/1
  Constant3/1 -> Data Type Conversion2/1
  FMS_In/1 -> Command_Mask/1(FMS_In), Bus Selector1/1
  Data Type Conversion/1 -> Bus Assignment/2
  Data Type Conversion1/1 -> Bus Assignment/3
  Constant1/1 -> Data Type Conversion/1
  Constant/1 -> Bus Assignment/1
  Data Type Conversion2/1 -> Bus Assignment/4
  Bus Selector1/3 -> Bus Assignment/7  "<u_cmd>"
  Bus Selector1/4 -> Bus Assignment/8  "<w_cmd>"
  Command_Mask/1(cmd_mask) -> Bus Assignment/9
  Bus Selector1/1 -> Bus Assignment/5  "<psi_rate_cmd>"
  Bus Selector1/2 -> Bus Assignment/6  "<theta_cmd>"

== system FMS/FMS Commander/Commander/Arm/Auto/Unknown ==
  Action Port : ActionPort  InitializeStates=reset  ActionType=default
  Bus Assignment : BusAssignment  AssignedSignals=reset,status,state,actuator_cmd
  Constant : Constant  Value=0  OutDataTypeStr=Bus: FMS_Out_Bus
  Constant1 : Constant  Value=VehicleStatus.Disarm
  Constant2 : Constant  OutDataTypeStr=Inherit: Inherit via back propagation
  Constant3 : Constant  Value=[1000;1000;1000;1000]  VectorParams1D=off  OutDataTypeStr=Inherit: Inherit via back propagation
  Constant4 : Constant  Value=zeros(12,1)  OutDataTypeStr=Inherit: Inherit via back propagation
  Constant5 : Constant  Value=VehicleState.Disarm
  Data Type Conversion : DataTypeConversion
  Data Type Conversion1 : DataTypeConversion
  Mux : Mux  Inputs=2
  FMS_Out : Outport
  wires:
  Mux/1 -> Bus Assignment/5
  Constant4/1 -> Mux/2
  Constant3/1 -> Mux/1
  Constant1/1 -> Data Type Conversion/1
  Constant2/1 -> Bus Assignment/2
  Bus Assignment/1 -> FMS_Out/1
  Constant/1 -> Bus Assignment/1
  Constant5/1 -> Data Type Conversion1/1
  Data Type Conversion/1 -> Bus Assignment/3
  Data Type Conversion1/1 -> Bus Assignment/4

== system FMS/FMS Commander/Commander/Arm/SubMode/Hold ==
  FMS_In : Inport
  Action Port : ActionPort  InitializeStates=reset  ActionType=case
      settings: CopyFcn=Stateflow.SLINSF.SimulinkMan.removeBlockPreDeleteFcn
  Bus Assignment : BusAssignment  AssignedSignals=status,state,ctrl_mode,u_cmd,ay_cmd,w_cmd
  Constant : Constant  Value=0  OutDataTypeStr=Bus: FMS_Out_Bus
  Constant1 : Constant  Value=VehicleState.Hold
  Constant2 : Constant  Value=ControlMode.POSCTL
  Constant3 : Constant  Value=0  OutDataTypeStr=Inherit: Inherit via back propagation
  Constant4 : Constant  Value=0  OutDataTypeStr=Inherit: Inherit via back propagation
  Constant5 : Constant  Value=VehicleStatus.Arm
  Constant6 : Constant  Value=0  OutDataTypeStr=Inherit: Inherit via back propagation
  Data Type Conversion : DataTypeConversion
  Data Type Conversion1 : DataTypeConversion
  Data Type Conversion2 : DataTypeConversion
  Terminator : Terminator
  FMS_Out : Outport
  wires:
  Bus Assignment/1 -> FMS_Out/1
  Constant/1 -> Bus Assignment/1
  Constant5/1 -> Data Type Conversion/1
  Data Type Conversion/1 -> Bus Assignment/2
  Constant1/1 -> Data Type Conversion1/1
  Data Type Conversion1/1 -> Bus Assignment/3
  Constant2/1 -> Data Type Conversion2/1
  Data Type Conversion2/1 -> Bus Assignment/4
  FMS_In/1 -> Terminator/1
  Constant3/1 -> Bus Assignment/5
  Constant4/1 -> Bus Assignment/6
  Constant6/1 -> Bus Assignment/7

== system FMS/FMS Commander/Commander/Arm/SubMode/Return ==
  FMS_In : Inport
  Action Port : ActionPort  InitializeStates=reset  ActionType=case
      settings: CopyFcn=Stateflow.SLINSF.SimulinkMan.removeBlockPreDeleteFcn
  Altitude Control : Subsystem
  Bus Assignment1 : BusAssignment  AssignedSignals=status,state,ctrl_mode,u_cmd,r_cmd,w_cmd
  Constant1 : Constant  Value=VehicleState.Return
  Constant2 : Constant  Value=0  OutDataTypeStr=Bus: FMS_Out_Bus
  Constant3 : Constant  Value=ControlMode.POSCTL
  Constant6 : Constant  Value=VehicleStatus.Arm
  Data Type Conversion : DataTypeConversion
  Data Type Conversion1 : DataTypeConversion
  Data Type Conversion2 : DataTypeConversion
  Position Command : Subsystem
  vel : Constant  Value=FMS_PARAM.CRUISE_SPEED  OutDataTypeStr=single
  FMS_Out : Outport
  wires:
  Constant3/1 -> Data Type Conversion2/1
  Constant2/1 -> Bus Assignment1/1
  Bus Assignment1/1 -> FMS_Out/1
  Data Type Conversion/1 -> Bus Assignment1/2
  Constant6/1 -> Data Type Conversion/1
  Data Type Conversion1/1 -> Bus Assignment1/3
  Data Type Conversion2/1 -> Bus Assignment1/4
  Constant1/1 -> Data Type Conversion1/1
  Position Command/1(r_cmd) -> Bus Assignment1/6
  FMS_In/1 -> Position Command/1(FMS_In), Altitude Control/1(FMS_In)
  vel/1 -> Bus Assignment1/5
  Altitude Control/1(w_cmd_mPs) -> Bus Assignment1/7

== system FMS/FMS Commander/Commander/Arm/SubMode/Unknown ==
  Action Port : ActionPort  InitializeStates=reset  ActionType=default
  Bus Assignment : BusAssignment  AssignedSignals=reset,status,state,actuator_cmd
  Constant : Constant  Value=0  OutDataTypeStr=Bus: FMS_Out_Bus
  Constant1 : Constant  Value=VehicleStatus.Disarm
  Constant2 : Constant  OutDataTypeStr=Inherit: Inherit via back propagation
  Constant3 : Constant  Value=[1000;1000;1000;1000]  VectorParams1D=off  OutDataTypeStr=Inherit: Inherit via back propagation
  Constant4 : Constant  Value=zeros(12,1)  OutDataTypeStr=Inherit: Inherit via back propagation
  Constant5 : Constant  Value=VehicleState.Disarm
  Data Type Conversion : DataTypeConversion
  Data Type Conversion1 : DataTypeConversion
  Mux : Mux  Inputs=2
  FMS_Out : Outport
  wires:
  Mux/1 -> Bus Assignment/5
  Constant4/1 -> Mux/2
  Constant3/1 -> Mux/1
  Constant1/1 -> Data Type Conversion/1
  Constant2/1 -> Bus Assignment/2
  Bus Assignment/1 -> FMS_Out/1
  Constant/1 -> Bus Assignment/1
  Constant5/1 -> Data Type Conversion1/1
  Data Type Conversion/1 -> Bus Assignment/3
  Data Type Conversion1/1 -> Bus Assignment/4

== system FMS/FMS Commander/Commander/Arm/Assist/Altitude/Altitude Command ==
  FMS_In : Inport
  Controller : Subsystem
  Detect Movement : Subsystem
  w_cmd_mPs : Outport
  wires:
  Detect Movement/1(motion_state) -> Controller/1(motion_state)
  FMS_In/1 -> Controller/2(FMS_In), Detect Movement/1(FMS_In)
  Controller/1(w_cmd_mPs) -> w_cmd_mPs/1

== system FMS/FMS Commander/Commander/Arm/Assist/Altitude/Heading Command ==
  FMS_In : Inport
  Bus Selector : BusSelector  OutputSignals=Pilot_Cmd.stick_roll
  DeadZone2 : Subsystem  mask{th=FMS_PARAM.ROLL_DZ}
      mask prompts: th "Threshold"
      mask Display: disp('Dead Zone')
  Gain6 : Gain  Gain=FMS_PARAM.MAX_R  OutDataTypeStr=single
  r_cmd : Outport
  wires:
  Bus Selector/1 -> DeadZone2/1(u)  "<stick_roll>"
  FMS_In/1 -> Bus Selector/1
  DeadZone2/1(y) -> Gain6/1
  Gain6/1 -> r_cmd/1

== system FMS/FMS Commander/Commander/Arm/Assist/Altitude/Speed Command ==
  FMS_In : Inport
  Bus Selector : BusSelector  OutputSignals=Pilot_Cmd.stick_pitch
  DeadZone2 : Subsystem  mask{th=FMS_PARAM.PITCH_DZ}
      mask prompts: th "Threshold"
      mask Display: disp('Dead Zone')
  Gain6 : Gain  Gain=FMS_PARAM.VEL_X_LIM  OutDataTypeStr=single
  u_cmd_radPs : Outport
  wires:
  Bus Selector/1 -> DeadZone2/1(u)  "<stick_pitch>"
  FMS_In/1 -> Bus Selector/1
  DeadZone2/1(y) -> Gain6/1
  Gain6/1 -> u_cmd_radPs/1

== system FMS/FMS Commander/Commander/Arm/Assist/Position/Altitude Command ==
  FMS_In : Inport
  Controller : Subsystem
  Detect Movement : Subsystem
  w_cmd_mPs : Outport
  wires:
  Detect Movement/1(motion_state) -> Controller/1(motion_state)
  FMS_In/1 -> Controller/2(FMS_In), Detect Movement/1(FMS_In)
  Controller/1(w_cmd_mPs) -> w_cmd_mPs/1

== system FMS/FMS Commander/Commander/Arm/Assist/Position/Heading Command ==
  FMS_In : Inport
  Bus Selector : BusSelector  OutputSignals=Pilot_Cmd.stick_roll
  DeadZone2 : Subsystem  mask{th=FMS_PARAM.ROLL_DZ}
      mask prompts: th "Threshold"
      mask Display: disp('Dead Zone')
  Gain6 : Gain  Gain=FMS_PARAM.MAX_R  OutDataTypeStr=single
  r_cmd : Outport
  wires:
  Bus Selector/1 -> DeadZone2/1(u)  "<stick_roll>"
  FMS_In/1 -> Bus Selector/1
  DeadZone2/1(y) -> Gain6/1
  Gain6/1 -> r_cmd/1

== system FMS/FMS Commander/Commander/Arm/Assist/Position/Speed Command ==
  FMS_In : Inport
  Controller : Subsystem
  Detect Movement : Subsystem
  u_cmd_radPs : Outport
  wires:
  FMS_In/1 -> Controller/2(FMS_In), Detect Movement/1(FMS_In)
  Detect Movement/1(motion_state) -> Controller/1(motion_state)
  Controller/1(uv_cmd_mPs) -> u_cmd_radPs/1

== system FMS/FMS Commander/Commander/Arm/Assist/Stabilize/Altitude Command  ==
  FMS_In : Inport
  Bus Selector : BusSelector  OutputSignals=Pilot_Cmd.stick_throttle
  DeadZone2 : Subsystem  mask{th=FMS_PARAM.THROTTLE_DZ}
      mask prompts: th "Threshold"
      mask Display: disp('Dead Zone')
  Gain6 : Gain  Gain=-FMS_PARAM.VEL_Z_LIM  OutDataTypeStr=single
  w_cmd_mPs : Outport
  wires:
  Bus Selector/1 -> DeadZone2/1(u)  "<stick_throttle>"
  FMS_In/1 -> Bus Selector/1
  DeadZone2/1(y) -> Gain6/1
  Gain6/1 -> w_cmd_mPs/1

== system FMS/FMS Commander/Commander/Arm/Assist/Stabilize/Heading Command ==
  FMS_In : Inport
  Bus Selector : BusSelector  OutputSignals=Pilot_Cmd.stick_roll
  DeadZone2 : Subsystem  mask{th=FMS_PARAM.ROLL_DZ}
      mask prompts: th "Threshold"
      mask Display: disp('Dead Zone')
  Gain6 : Gain  Gain=FMS_PARAM.MAX_R  OutDataTypeStr=single
  r_cmd : Outport
  wires:
  Bus Selector/1 -> DeadZone2/1(u)  "<stick_roll>"
  FMS_In/1 -> Bus Selector/1
  DeadZone2/1(y) -> Gain6/1
  Gain6/1 -> r_cmd/1

== system FMS/FMS Commander/Commander/Arm/Assist/Stabilize/Speed Command ==
  FMS_In : Inport
  Bus Selector : BusSelector  OutputSignals=Pilot_Cmd.stick_pitch
  DeadZone2 : Subsystem  mask{th=FMS_PARAM.PITCH_DZ}
      mask prompts: th "Threshold"
      mask Display: disp('Dead Zone')
  Gain6 : Gain  Gain=FMS_PARAM.VEL_X_LIM  OutDataTypeStr=single
  u_cmd_radPs : Outport
  wires:
  Bus Selector/1 -> DeadZone2/1(u)  "<stick_pitch>"
  FMS_In/1 -> Bus Selector/1
  DeadZone2/1(y) -> Gain6/1
  Gain6/1 -> u_cmd_radPs/1

== system FMS/FMS Commander/Commander/Arm/Auto/Mission/Mission_SubSystem ==
  FMS_In : Inport
  Reset : ResetPort  DisableCoverage=on
  Altitude Control : Subsystem
  Bus Assignment : BusAssignment  AssignedSignals=status,state,ctrl_mode,u_cmd,r_cmd,w_cmd
  Constant : Constant  Value=0  OutDataTypeStr=Bus: FMS_Out_Bus
  Constant1 : Constant  Value=VehicleStatus.Arm
  Constant2 : Constant  Value=VehicleState.Mission
  Constant3 : Constant  Value=ControlMode.POSCTL
  Data Type Conversion : DataTypeConversion
  Data Type Conversion1 : DataTypeConversion
  Data Type Conversion2 : DataTypeConversion
  Position Command : Subsystem
  vel : Constant  Value=FMS_PARAM.CRUISE_SPEED  OutDataTypeStr=single
  FMS_Out : Outport
  wires:
  Data Type Conversion1/1 -> Bus Assignment/3
  Constant1/1 -> Data Type Conversion/1
  Data Type Conversion2/1 -> Bus Assignment/4
  Data Type Conversion/1 -> Bus Assignment/2
  Constant2/1 -> Data Type Conversion1/1
  Constant3/1 -> Data Type Conversion2/1
  Constant/1 -> Bus Assignment/1
  Bus Assignment/1 -> FMS_Out/1
  vel/1 -> Bus Assignment/5
  FMS_In/1 -> Altitude Control/1(FMS_In), Position Command/1(FMS_In)
  Position Command/1(r_cmd) -> Bus Assignment/6
  Altitude Control/1(w_cmd_mPs) -> Bus Assignment/7

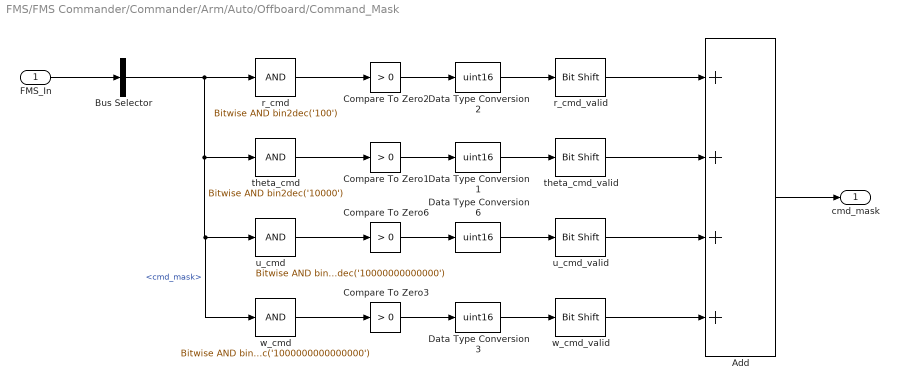
== system FMS/FMS Commander/Commander/Arm/Auto/Offboard/Command_Mask ==
  FMS_In : Inport
  Add : Sum  Inputs=++++
  Bus Selector : BusSelector  OutputSignals=Auto_Cmd.cmd_mask
  Compare To Zero{1..3,6} (4 alike) : simulink/Logic and Bit Operations/Compare To Zero  relop=>  OutDataTypeStr=boolean
  Data Type Conversion{1..3,6} (4 alike) : DataTypeConversion  OutDataTypeStr=uint16
  r_cmd : simulink/Logic and Bit Operations/Bitwise Operator  logicop=AND  UseBitMask=on  BitMask=bin2dec('100')  BitMaskRealWorld=Stored Integer
  r_cmd_valid : hdlsllib/Logic and Bit Operations/Bit Shift  mode=Shift Left Logical  N=2
      settings: SourceProductName=HDL Coder  SourceProductBaseCode=HD
  theta_cmd : simulink/Logic and Bit Operations/Bitwise Operator  logicop=AND  UseBitMask=on  BitMask=bin2dec('10000')  BitMaskRealWorld=Stored Integer
  theta_cmd_valid : hdlsllib/Logic and Bit Operations/Bit Shift  mode=Shift Left Logical  N=4
      settings: SourceProductName=HDL Coder  SourceProductBaseCode=HD
  u_cmd : simulink/Logic and Bit Operations/Bitwise Operator  logicop=AND  UseBitMask=on  BitMask=bin2dec('10000000000000')  BitMaskRealWorld=Stored Integer
  u_cmd_valid : hdlsllib/Logic and Bit Operations/Bit Shift  mode=Shift Left Logical  N=6
      settings: SourceProductName=HDL Coder  SourceProductBaseCode=HD
  w_cmd : simulink/Logic and Bit Operations/Bitwise Operator  logicop=AND  UseBitMask=on  BitMask=bin2dec('1000000000000000')  BitMaskRealWorld=Stored Integer
  w_cmd_valid : hdlsllib/Logic and Bit Operations/Bit Shift  mode=Shift Left Logical  N=8
      settings: SourceProductName=HDL Coder  SourceProductBaseCode=HD
  cmd_mask : Outport
  wires:
  FMS_In/1 -> Bus Selector/1
  r_cmd/1 -> Compare To Zero2/1
  Compare To Zero2/1 -> Data Type Conversion2/1
  Data Type Conversion2/1 -> r_cmd_valid/1
  Bus Selector/1 -> w_cmd/1, u_cmd/1, theta_cmd/1, r_cmd/1  "<cmd_mask>"
  Add/1 -> cmd_mask/1
  Data Type Conversion6/1 -> u_cmd_valid/1
  Compare To Zero6/1 -> Data Type Conversion6/1
  u_cmd/1 -> Compare To Zero6/1
  Data Type Conversion1/1 -> theta_cmd_valid/1
  Compare To Zero1/1 -> Data Type Conversion1/1
  theta_cmd/1 -> Compare To Zero1/1
  w_cmd/1 -> Compare To Zero3/1
  Data Type Conversion3/1 -> w_cmd_valid/1
  Compare To Zero3/1 -> Data Type Conversion3/1
  r_cmd_valid/1 -> Add/1
  u_cmd_valid/1 -> Add/3
  theta_cmd_valid/1 -> Add/2
  w_cmd_valid/1 -> Add/4

== system FMS/FMS Commander/Commander/Arm/SubMode/Return/Altitude Control ==
  FMS_In : Inport
  Bus Selector3 : BusSelector  OutputSignals=INS_Out.h_R
  Gain : Gain  Gain=FMS_PARAM.Z_P
  Saturation1 : Saturate  UpperLimit=FMS_PARAM.VEL_Z_LIM  LowerLimit=-FMS_PARAM.VEL_Z_LIM
  Sum2 : Sum  Inputs=|+-
  Target Height : Subsystem
  w_cmd_mPs : Outport
  wires:
  FMS_In/1 -> Bus Selector3/1, Target Height/1(FMS_In)
  Bus Selector3/1 -> Sum2/1  "<h_R>"
  Sum2/1 -> Gain/1
  Gain/1 -> Saturation1/1
  Target Height/1(h_R_sp) -> Sum2/2  "h_R_sp"
  Saturation1/1 -> w_cmd_mPs/1

== system FMS/FMS Commander/Commander/Arm/SubMode/Return/Position Command ==
  FMS_In : Inport
  L1 : Constant  Value=FMS_PARAM.L1  OutDataTypeStr=single
  Velocity Commander : Subsystem
  Way Points : Subsystem
  r_cmd : Outport
  wires:
  FMS_In/1 -> Velocity Commander/5(FMS_In), Way Points/1(FMS_In)
  Way Points/3(p3) -> Velocity Commander/3(p3)
  Velocity Commander/1(r_cmd) -> r_cmd/1
  Way Points/1(p1) -> Velocity Commander/1(p1)
  L1/1 -> Velocity Commander/4(L1)
  Way Points/2(p2) -> Velocity Commander/2(p2)

== system FMS/FMS Commander/Commander/Arm/Assist/Altitude/Altitude Command/Controller ==
  motion_state : Inport
  In Bus Element : Inport  Port=2  PortName=FMS_In
  In Bus Element1 : Inport  Port=2  PortName=FMS_In
  Brake Control : Subsystem  TreatAsAtomicUnit=on
  Hold Control : Subsystem  TreatAsAtomicUnit=on
  Merge : Merge  Inputs=3
  Move Control : Subsystem  TreatAsAtomicUnit=on
  Saturation1 : Saturate  UpperLimit=FMS_PARAM.VEL_Z_LIM  LowerLimit=-FMS_PARAM.VEL_Z_LIM
  Switch Case : SwitchCase  CaseConditions={MotionState.Hold, MotionState.Brake, MotionState.Move}  ShowDefaultCase=off
  w_cmd_mPs : Outport
  wires:
  Move Control/1(w_cmd_mPs) -> Merge/3
  Brake Control/1(w_cmd_mPs) -> Merge/2
  Hold Control/1(w_cmd_mPs) -> Merge/1
  In Bus Element/1 -> Hold Control/1(FMS_In)
  Switch Case/2 -> Brake Control/Action
  Switch Case/1 -> Hold Control/Action
  motion_state/1 -> Switch Case/1
  Saturation1/1 -> w_cmd_mPs/1
  Merge/1 -> Saturation1/1
  Switch Case/3 -> Move Control/Action
  In Bus Element1/1 -> Move Control/1(FMS_In)

== system FMS/FMS Commander/Commander/Arm/Assist/Altitude/Altitude Command/Detect Movement ==
  FMS_In : Inport
  Abs : Abs
  Abs1 : Abs
  Bus Selector : BusSelector  OutputSignals=Pilot_Cmd.stick_throttle,INS_Out.vd
  Compare To Constant : simulink/Logic and Bit Operations/Compare To Constant  relop=>  const=FMS_PARAM.THROTTLE_DZ  OutDataTypeStr=boolean
  Motion Status : Stateflow chart  TreatAsAtomicUnit=on
  motion_state : Outport
  wires:
  FMS_In/1 -> Bus Selector/1
  Abs1/1 -> Compare To Constant/1
  Motion Status/1(state) -> motion_state/1
  Compare To Constant/1 -> Motion Status/1(motion_req)
  Abs/1 -> Motion Status/2(speed)
  Bus Selector/1 -> Abs1/1  "<stick_throttle>"
  Bus Selector/2 -> Abs/1  "<vd>"

== system FMS/FMS Commander/Commander/Arm/Assist/Altitude/Heading Command/DeadZone2 ==
  u : Inport
  Dead Zone : DeadZone  LowerValue=-th  UpperValue=th  SaturateOnIntegerOverflow=on
  Gain : Gain  Gain=1/(1-th)
  y : Outport
  wires:
  u/1 -> Dead Zone/1
  Dead Zone/1 -> Gain/1
  Gain/1 -> y/1

== system FMS/FMS Commander/Commander/Arm/Assist/Altitude/Speed Command/DeadZone2 ==
  u : Inport
  Dead Zone : DeadZone  LowerValue=-th  UpperValue=th  SaturateOnIntegerOverflow=on
  Gain : Gain  Gain=1/(1-th)
  y : Outport
  wires:
  u/1 -> Dead Zone/1
  Dead Zone/1 -> Gain/1
  Gain/1 -> y/1

== system FMS/FMS Commander/Commander/Arm/Assist/Position/Altitude Command/Controller ==
  motion_state : Inport
  In Bus Element : Inport  Port=2  PortName=FMS_In
  In Bus Element1 : Inport  Port=2  PortName=FMS_In
  Brake Control : Subsystem  TreatAsAtomicUnit=on
  Hold Control : Subsystem  TreatAsAtomicUnit=on
  Merge : Merge  Inputs=3
  Move Control : Subsystem  TreatAsAtomicUnit=on
  Saturation1 : Saturate  UpperLimit=FMS_PARAM.VEL_Z_LIM  LowerLimit=-FMS_PARAM.VEL_Z_LIM
  Switch Case : SwitchCase  CaseConditions={MotionState.Hold, MotionState.Brake, MotionState.Move}  ShowDefaultCase=off
  w_cmd_mPs : Outport
  wires:
  Move Control/1(w_cmd_mPs) -> Merge/3
  Brake Control/1(w_cmd_mPs) -> Merge/2
  Hold Control/1(w_cmd_mPs) -> Merge/1
  In Bus Element/1 -> Hold Control/1(FMS_In)
  Switch Case/2 -> Brake Control/Action
  Switch Case/1 -> Hold Control/Action
  motion_state/1 -> Switch Case/1
  Saturation1/1 -> w_cmd_mPs/1
  Merge/1 -> Saturation1/1
  Switch Case/3 -> Move Control/Action
  In Bus Element1/1 -> Move Control/1(FMS_In)
